simulink subsystem "pieromfsZ"  (R2022b)
settings: Solver=VariableStepAuto  StartTime=0.0  StopTime=10.0  RelTol=1e-3
settings Model: Creator=miriamfreiriasanjuan  LastModifiedBy=miriamfreiriasanjuan

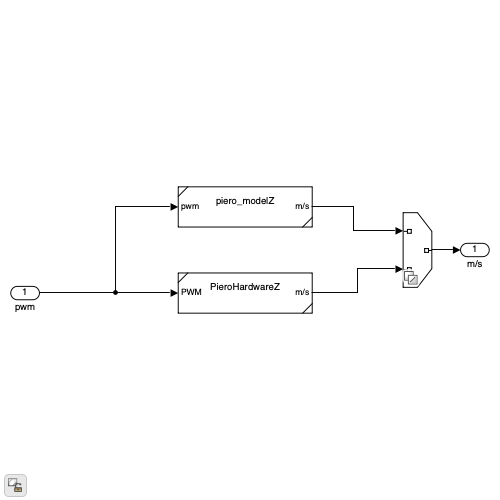
[thumbnail: Simulink's stored preview of the top-level diagram]
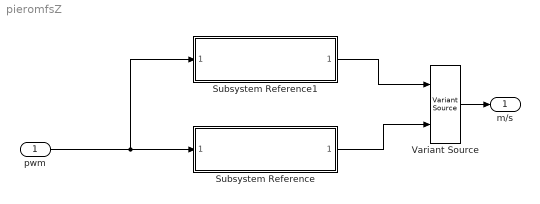
== system pieromfsZ ==
  pwm : Inport
  Subsystem Reference : Subsystem  ReferencedSubsystem=PieroHardwareZ
  Subsystem Reference1 : Subsystem  ReferencedSubsystem=piero_modelZ
  Variant Source : VariantSource  VariantControlMode=sim codegen switching
  m/s : Outport
  wires:
  Variant Source/1 -> m/s/1
  pwm/1 -> Subsystem Reference/1, Subsystem Reference1/1
  Subsystem Reference1/1 -> Variant Source/1
  Subsystem Reference/1 -> Variant Source/2
